simulink model "Hexalock.slx"  (R2026b)
settings: Solver=VariableStepAuto  StopTime=inf
undefined symbols (not defined in the file): gray
(part 5 of 5)

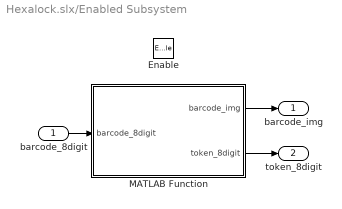
== system Hexalock.slx/Enabled Subsystem ==
  barcode_8digit : Inport
  Enable : EnablePort
  MATLAB Function : MATLAB Function  TreatAsAtomicUnit=on
  barcode_img : Outport  InitialOutput=uint8(255 * ones(80, 320))
  token_8digit : Outport  Port=2  InitialOutput=0
  wires:
  MATLAB Function/1(barcode_img) -> barcode_img/1
  MATLAB Function/2(token_8digit) -> token_8digit/1
  barcode_8digit/1 -> MATLAB Function/1(barcode_8digit)

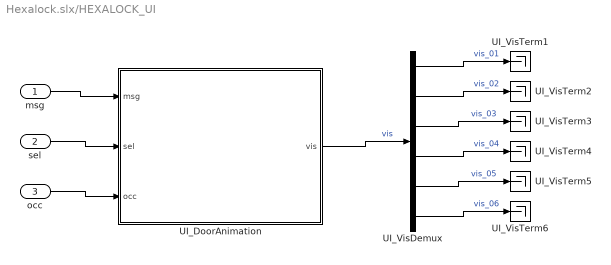
== system Hexalock.slx/HEXALOCK_UI ==
  msg : Inport
  sel : Inport  Port=2
  occ : Inport  Port=3
  UI_DoorAnimation : Stateflow chart  TreatAsAtomicUnit=on
  UI_VisDemux : Demux  Outputs=6
  UI_VisTerm{1..6} (6 alike) : Terminator
  wires:
  msg/1 -> UI_DoorAnimation/1(msg)
  sel/1 -> UI_DoorAnimation/2(sel)
  occ/1 -> UI_DoorAnimation/3(occ)
  UI_DoorAnimation/1(vis) -> UI_VisDemux/1  "vis"
  UI_VisDemux/1 -> UI_VisTerm1/1  "vis_01"
  UI_VisDemux/2 -> UI_VisTerm2/1  "vis_02"
  UI_VisDemux/3 -> UI_VisTerm3/1  "vis_03"
  UI_VisDemux/4 -> UI_VisTerm4/1  "vis_04"
  UI_VisDemux/5 -> UI_VisTerm5/1  "vis_05"
  UI_VisDemux/6 -> UI_VisTerm6/1  "vis_06"

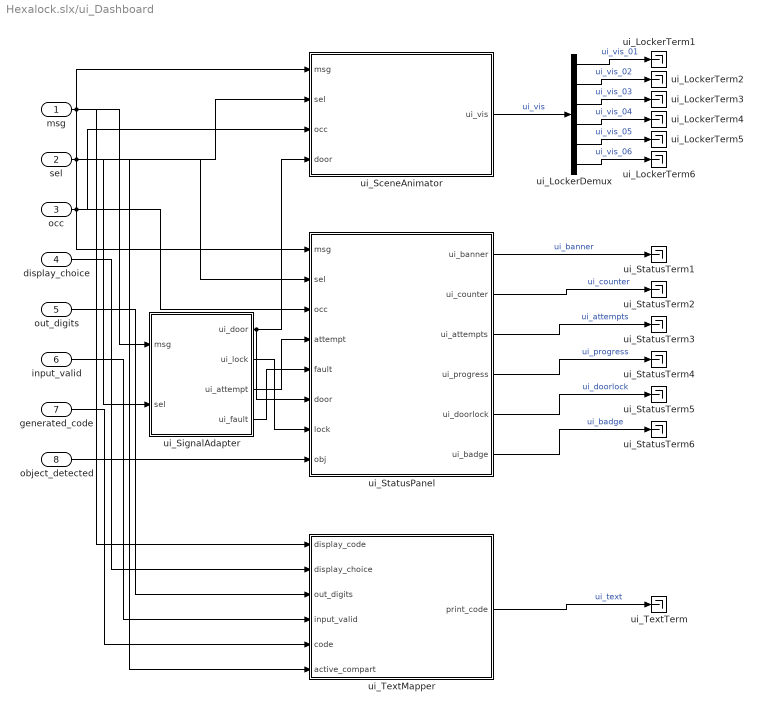
== system Hexalock.slx/ui_Dashboard ==
  msg : Inport
  sel : Inport  Port=2
  occ : Inport  Port=3
  display_choice : Inport  Port=4
  out_digits : Inport  Port=5
  input_valid : Inport  Port=6
  generated_code : Inport  Port=7
  object_detected : Inport  Port=8
  ui_LockerDemux : Demux  Outputs=6
  ui_LockerTerm{1..6} (6 alike) : Terminator
  ui_SceneAnimator : Stateflow chart  TreatAsAtomicUnit=on
  ui_SignalAdapter : Stateflow chart  TreatAsAtomicUnit=on
  ui_StatusPanel : Stateflow chart  TreatAsAtomicUnit=on
  ui_StatusTerm{1..6} (6 alike) : Terminator
  ui_TextMapper : MATLAB Function  TreatAsAtomicUnit=on
  ui_TextTerm : Terminator
  wires:
  msg/1 -> ui_SignalAdapter/1(msg), ui_SceneAnimator/1(msg), ui_StatusPanel/1(msg), ui_TextMapper/1(display_code)
  sel/1 -> ui_SignalAdapter/2(sel), ui_SceneAnimator/2(sel), ui_StatusPanel/2(sel), ui_TextMapper/6(active_compart)
  occ/1 -> ui_SceneAnimator/3(occ), ui_StatusPanel/3(occ)
  ui_SignalAdapter/1(ui_door) -> ui_SceneAnimator/4(door), ui_StatusPanel/6(door)
  ui_SceneAnimator/1(ui_vis) -> ui_LockerDemux/1  "ui_vis"
  ui_LockerDemux/1 -> ui_LockerTerm1/1  "ui_vis_01"
  ui_LockerDemux/2 -> ui_LockerTerm2/1  "ui_vis_02"
  ui_LockerDemux/3 -> ui_LockerTerm3/1  "ui_vis_03"
  ui_LockerDemux/4 -> ui_LockerTerm4/1  "ui_vis_04"
  ui_LockerDemux/5 -> ui_LockerTerm5/1  "ui_vis_05"
  ui_LockerDemux/6 -> ui_LockerTerm6/1  "ui_vis_06"
  ui_SignalAdapter/3(ui_attempt) -> ui_StatusPanel/4(attempt)
  ui_SignalAdapter/4(ui_fault) -> ui_StatusPanel/5(fault)
  ui_SignalAdapter/2(ui_lock) -> ui_StatusPanel/7(lock)
  object_detected/1 -> ui_StatusPanel/8(obj)
  ui_StatusPanel/1(ui_banner) -> ui_StatusTerm1/1  "ui_banner"
  ui_StatusPanel/2(ui_counter) -> ui_StatusTerm2/1  "ui_counter"
  ui_StatusPanel/3(ui_attempts) -> ui_StatusTerm3/1  "ui_attempts"
  ui_StatusPanel/4(ui_progress) -> ui_StatusTerm4/1  "ui_progress"
  ui_StatusPanel/5(ui_doorlock) -> ui_StatusTerm5/1  "ui_doorlock"
  ui_StatusPanel/6(ui_badge) -> ui_StatusTerm6/1  "ui_badge"
  display_choice/1 -> ui_TextMapper/2(display_choice)
  out_digits/1 -> ui_TextMapper/3(out_digits)
  input_valid/1 -> ui_TextMapper/4(input_valid)
  generated_code/1 -> ui_TextMapper/5(code)
  ui_TextMapper/1(print_code) -> ui_TextTerm/1  "ui_text"

== matlab function Hexalock.slx/Enabled Subsystem/MATLAB Function ==
  data: barcode_8digit input; barcode_img output; token_8digit output double size=1

function [barcode_img, token_8digit] = Barcode_Generator(barcode_8digit)
% Generate a Code 128C barcode for an 8-digit locker token.
% Fixed-size grayscale image: 80 rows x 320 columns.
% 0 = black, 255 = white.

barcode_img = uint8(255 * ones(80, 320));
token_8digit = barcode_8digit;
digits = zeros(1, 8);
temp = token_8digit;

for i = 8:-1:1
    digits(i) = mod(temp, 10);
    temp = floor(temp / 10);
end

% Code 128C encodes two digits per symbol.
pairs = zeros(1, 4);

for i = 1:4
    pairs(i) = digits(2*i-1)*10 + digits(2*i);
end

% Code 128 symbol patterns.
% Each row contains six alternating bar/space widths.
% Rows 1-106 correspond to symbol values 0-105.
patterns = uint8([
    2 1 2 2 2 2;
    2 2 2 1 2 2;
    2 2 2 2 2 1;
    1 2 1 2 2 3;
    1 2 1 3 2 2;
    1 3 1 2 2 2;
    1 2 2 2 1 3;
    1 2 2 3 1 2;
    1 3 2 2 1 2;
    2 2 1 2 1 3;
    2 2 1 3 1 2;
    2 3 1 2 1 2;
    1 1 2 2 3 2;
    1 2 2 1 3 2;
    1 2 2 2 3 1;
    1 1 3 2 2 2;
    1 2 3 1 2 2;
    1 2 3 2 2 1;
    2 2 3 2 1 1;
    2 2 1 1 3 2;
    2 2 1 2 3 1;
    2 1 3 2 1 2;
    2 2 3 1 1 2;
    3 1 2 1 3 1;
    3 1 1 2 2 2;
    3 2 1 1 2 2;
    3 2 1 2 2 1;
    3 1 2 2 1 2;
    3 2 2 1 1 2;
    3 2 2 2 1 1;
    2 1 2 1 2 3;
    2 1 2 3 2 1;
    2 3 2 1 2 1;
    1 1 1 3 2 3;
    1 3 1 1 2 3;
    1 3 1 3 2 1;
    1 1 2 3 1 3;
    1 3 2 1 1 3;
    1 3 2 3 1 1;
    2 1 1 3 1 3;
    2 3 1 1 1 3;
    2 3 1 3 1 1;
    1 1 2 1 3 3;
    1 1 2 3 3 1;
    1 3 2 1 3 1;
    1 1 3 1 2 3;
    1 1 3 3 2 1;
    1 3 3 1 2 1;
    3 1 3 1 2 1;
    2 1 1 3 3 1;
    2 3 1 1 3 1;
    2 1 3 1 1 3;
    2 1 3 3 1 1;
    2 1 3 1 3 1;
    3 1 1 1 2 3;
    3 1 1 3 2 1;
    3 3 1 1 2 1;
    3 1 2 1 1 3;
    3 1 2 3 1 1;
    3 3 2 1 1 1;
    3 1 4 1 1 1;
    2 2 1 4 1 1;
    4 3 1 1 1 1;
    1 1 1 2 2 4;
    1 1 1 4 2 2;
    1 2 1 1 2 4;
    1 2 1 4 2 1;
    1 4 1 1 2 2;
    1 4 1 2 2 1;
    1 1 2 2 1 4;
    1 1 2 4 1 2;
    1 2 2 1 1 4;
    1 2 2 4 1 1;
    1 4 2 1 1 2;
    1 4 2 2 1 1;
    2 4 1 2 1 1;
    2 2 1 1 1 4;
    4 1 3 1 1 1;
    2 4 1 1 1 2;
    1 3 4 1 1 1;
    1 1 1 2 4 2;
    1 2 1 1 4 2;
    1 2 1 2 4 1;
    1 1 4 2 1 2;
    1 2 4 1 1 2;
    1 2 4 2 1 1;
    4 1 1 2 1 2;
    4 2 1 1 1 2;
    4 2 1 2 1 1;
    2 1 2 1 4 1;
    2 1 4 1 2 1;
    4 1 2 1 2 1;
    1 1 1 1 4 3;
    1 1 1 3 4 1;
    1 3 1 1 4 1;
    1 1 4 1 1 3;
    1 1 4 3 1 1;
    4 1 1 1 1 3;
    4 1 1 3 1 1;
    1 1 3 1 4 1;
    1 1 4 1 3 1;
    3 1 1 1 4 1;
    4 1 1 1 3 1;
    2 1 1 4 1 2;
    2 1 1 2 1 4;
    2 1 1 2 3 2
]);

% Start Code C = 105.
% Checksum = (105 + weighted data symbols) mod 103.
checksum = 105;

for i = 1:4
    checksum = checksum + i * pairs(i);
end

checksum = mod(checksum, 103);

% Complete symbol sequence:
% Start C, 4 data pairs, checksum.
symbols = [105 pairs checksum];

% Fixed output width: 320 pixels.
% Each module is 2 pixels wide.
% Code 128C: 90 modules including stop.
% Left quiet zone begins at pixel 61.
module_width = 2;
x = 61;

% Draw six normal Code 128 symbols.
for s = 1:6
    symbol_value = symbols(s);
    widths = patterns(symbol_value + 1, :);

    for k = 1:6
        pixel_width = double(widths(k)) * module_width;

        % Odd positions represent black bars.
        if mod(k, 2) == 1
            barcode_img(9:72, x:x+pixel_width-1) = 0;
        end

        x = x + pixel_width;
    end
end

% Standard Code 128 stop pattern: 2331112.
stop_widths = [2 3 3 1 1 1 2];

for k = 1:7
    pixel_width = stop_widths(k) * module_width;

    if mod(k, 2) == 1
        barcode_img(9:72, x:x+pixel_width-1) = 0;
    end

    x = x + pixel_width;
end

end

== matlab function Hexalock.slx/MATLAB Function ==
  data: display_code input; print_code output; display_choice input; out_digits input; input_valid input; code input double size=1; active_compart input
function print_code = DisplayMapper(display_code, display_choice, out_digits, input_valid, code, active_compart)
% 1. Base prompt mapping based on system state
switch display_code
    % --- System / Idle ---
    case 0
        base_msg = "Welcome! 1#: Store | 2#: Retrieve | 333#: Maintenance";
    case 5
        base_msg = "Session timeout! Please start again";
    case 8
        base_msg = "Fault detected! Please wait for maintenance";
    case 11
        base_msg = "System locked: Attempt limit exceeded";

        % --- Store Parcel Flow ---
    case 1
        base_msg = "Select locker (1-6) + #";
    case 2
        base_msg = "Sorry, compartment unavailable";
    case 4
        base_msg = "Please place parcel";
    case 7
        base_msg = "Parcel stored! Please collect your receipt. Password:" + string(code);
    case 17
        base_msg = "Storage unavailable. All compartments are full.Please click # to return to main screen";

        % --- Retrieve Parcel Flow ---
    case 16
        base_msg = "Retrieval unavailable. All compartments are empty.Please click # to return to main screen";
    case 9
        base_msg = "Enter 6-digit PIN + #";
    case 10
        base_msg = "Error: Wrong PIN (6 digits), try again";
    case 12
        base_msg = "Please collect your parcel";
    case 13
        base_msg = "Parcel collected successfully!";
    case 26
        base_msg = "Retrieve: 11# Scan barcode | 22# Enter PIN";
    case 27
        base_msg = "Please scan your barcode";
    case 28
        base_msg = "Error: Barcode not recognised, try again";

        % --- Open & Close ---
    case 3
        base_msg = "Door " + active_compart + " opening";
    case 6
        base_msg = "Door Closing";

        % --- Maintenance Mode ---
    case 14
        base_msg = "Confirm authorisation";
    case 15
        base_msg = "To exit: confirm authorisation";
    case 18
        base_msg = "Enter Maintenance Id";
    case 19
        base_msg = "Enter Maintenance Pin";
    case 20
        base_msg = "Maintenance ID error";
    case 21
        base_msg = "Maintenance PIN error";
    case 22
        base_msg = "Maintenance Entry Successful";
    case 23
        base_msg = "MAINT ACTIVE: 1-6# Clear Box | 9# Reset All | 999# Exit";
    case 24
        base_msg = "Admin: Compartment Cleared";
    case 25
        base_msg = "Admin: All Compartments Reset!";


        % --- Default Fallback ---
    otherwise   % state 16
        base_msg = "System Ready";
end

% 2. Dynamic display rendering with input stream
if input_valid == 1
    % Instant feedback when '#' is pressed
    if out_digits > 0
        num_str = sprintf('%0*d', int64(out_digits), int64(display_choice));
        print_code = base_msg + "  [OK: " + num_str + "]";
    else
        print_code = base_msg + "  [Confirmed]";
    end

elseif out_digits > 0
    % Active typing stage: append real-time 1 to 6 digit inputs
    num_str = sprintf('%0*d', int64(out_digits), int64(display_choice));
    print_code = base_msg + "  [Input: " + num_str + "]";

else
    % Default idle or after '*' is pressed (out_digits == 0): restore clean prompt immediately
    print_code = base_msg;
end
end

== stateflow chart Hexalock.slx/Chart ==
  state Controller [parallel]
    settings: executionOrder=1
    state Main
      state StoreParcel
        state DisplayAvailable
        state OpenDoor
          en:
          lock(active_compart) = 0;
          lock_sensor(active_compart) = 0;
          motor(active_compart) = 0;
          door_sensor(active_compart) = 1;
          du:
          %Stop the motor if a fault has been detected
          if fault_detected == 1
          motor(active_compart) = 0;
          %If unlocking takes too long, stop motor and detect fault
          elseif elapsed(sec) >= 5 && ...
          lock_sensor(active_compart) ~= 0
          motor(active_compart) = 0;
          fault_detected = 1;
          %When door succesfully opens
          elseif door_sensor(active_compart) == 1
          motor(active_compart) = 0;
          %Fault detection check
          elseif door_sensor(active_compart) == 0 ||...
          lock_sensor(active_compart) == 1 ||...
          motor(active_compart) == 1;
          fault_detected = 1;
          %If it takes too long to open the door, detect fault
          elseif elapsed(sec) >= 15
          motor(active_compart) = 0;
          fault_detected = 1;
          %Turn the motor on, only after unlocking
          elseif lock_sensor(active_compart) == 0 && door_sensor(active_compart) == 0
          motor(active_compart) = 1;
          end
        state SelectCompartment
          en:
          active_compart = 0;
          du:
          if input_valid == 1 && display_choice >= 1 && display_choice <= 6
          active_compart = display_choice;
          %If locker is full, show relevant message
          if db_occupied(active_compart) == true
          outputMessage = 2;
          end
          end
        state TimeoutCloseDoor
          en:
          motor(active_compart) = -1;
          lock(active_compart) = 1;
          lock_sensor(active_compart) = 1;
          door_sensor(active_compart) = 0;
          du:
          % Stop motor if fault detected
          if fault_detected == 1
          motor(active_compart) = 0;
          %If door doesn't shut, stop motor and detect fault
          elseif elapsed(sec) >= 10 && ...
          door_sensor(active_compart) ~= 0
          motor(active_compart) = 0;
          fault_detected = 1;
          %if door is shut, stop motor and lock
          elseif door_sensor(active_compart) == 0
          motor(active_compart) = 0;
          lock(active_compart) = 1;
          %Fault detection check
          elseif door_sensor(active_compart) == 1 ||...
          lock_sensor(active_compart) == 0 ||...
          motor(active_compart) == 0;
          fault_detected = 1;
          end
          %If locking takes too long, detect fault
          if elapsed(sec) >= 5 && ...
          door_sensor(active_compart) == 0 && ...
          lock_sensor(active_compart) ~= 1
          fault_detected = 1;
          end
        state WaitForParcel
        state CloseDoor
          en:
          motor(active_compart) = -1;
          lock(active_compart) = 1;
          lock_sensor(active_compart) = 1;
          door_sensor(active_compart) = 0;
          object_sensor(active_compart) = 1;
          du:
          %Stop the motor and lock the door is closed
          if door_sensor(active_compart) == 0
          motor(active_compart) = 0;
          lock(active_compart) = 1;
          elseif door_sensor(active_compart) == 1 ||...
          lock_sensor(active_compart) == 0 ||...
          motor(active_compart) == 0;
          fault_detected = 1;
          end
          %If door doesn't shut, stop motor and detect fault
          if elapsed(sec) >= 10 && ...
          door_sensor(active_compart) ~= 0
          motor(active_compart) = 0;
          fault_detected = 1;
          outputMessage = 6;
          end
          %If locking takes too long, detect fault
          if elapsed(sec) >= 15 && ...
          door_sensor(active_compart) == 0 && ...
          lock_sensor(active_compart) ~= 1
          fault_detected = 1;
          end
          % Stop motor if fault detected
          if fault_detected == 1
          motor(active_compart) = 0;
          end
        state CheckPIN
          en:
          pin_candidate = double(random_pin);
          du:
          %Ensure the PIN isn't already used by an occupied locker in the DB
          if any((db_pins == pin_candidate) & db_occupied)
          pin_candidate = pin_candidate + 1;
          if pin_candidate > 999999
          pin_candidate = 100000;
          end
          end
        state StorageComplete
        (default) -> DisplayAvailable
        DisplayAvailable -> SelectCompartment : {outputMessage = 1;}
        SelectCompartment -> DisplayAvailable [order 1] : [after(5, sec) && active_compart >= 1 && active_compart <= 6 && ...
            |  db_occupied(active_compart) == true]
        SelectCompartment -> Controller.Main.StoreParcel.OpenDoor [order 2] : [active_compart >= 1 && active_compart <= 6 && ...
            |  db_occupied(active_compart) == false]{outputMessage = 3;}
        Controller.Main.StoreParcel.OpenDoor -> WaitForParcel : [after(2,sec) && door_sensor(active_compart) == 1 && ...
            |  lock_sensor(active_compart) == 0 && ...
            |  motor(active_compart) == 0 && ...
            |  fault_detected == 0]{outputMessage = 4;}
        WaitForParcel -> Controller.Main.StoreParcel.TimeoutCloseDoor [order 2] : [after(5,sec)]{outputMessage = 5;}
        WaitForParcel -> Controller.Main.StoreParcel.CloseDoor [order 1] : [object_detected == 1]{outputMessage = 6;}
        Controller.Main.StoreParcel.CloseDoor -> CheckPIN : [after(2,sec) && ...
            |  door_sensor(active_compart) == 0 && ...
            |  lock_sensor(active_compart) == 1 && ...
            |  motor(active_compart) == 0 && ...
            |  fault_detected == 0]
        CheckPIN -> StorageComplete : [~any((db_pins == pin_candidate) & db_occupied) && ...
            |  fault_detected == 0 && ...
            |  door_sensor(active_compart) == 0 && ...
            |  lock_sensor(active_compart) == 1 && ...
            |  motor(active_compart) == 0]
            | {generated_code = pin_candidate;
            |  store_req = true;
            |  outputMessage = 7;}
        Controller.Main.StoreParcel.TimeoutCloseDoor -> StorageComplete : [after(2, sec) && door_sensor(active_compart) == 0 && ...
            |  lock_sensor(active_compart) == 1 && ...
            |  motor(active_compart) == 0 && ...
            |  fault_detected == 0]{outputMessage = 6;}
      state Idle
        en:
        % Reset counters and selections for next user
        attempt = 0;
        active_compart = 0;
        compart_found = 0;
        fault_detected = 0;
        % Fail safe hardware enforcement
        motor = [0, 0, 0, 0, 0, 0];
        lock_sensor = [1, 1, 1, 1, 1, 1];
        door_sensor = [0, 0, 0, 0, 0, 0];
        %Display message
        outputMessage = 0;
        du:
        % Check the database: all empty = cannot retrieve, all full = cannot store
        if input_valid == 1 && display_choice == 2 && ~any(db_occupied)
        outputMessage = 16;
        elseif input_valid == 1 && display_choice == 1 && all(db_occupied)
        outputMessage = 17;
        elseif input_valid == 1
        outputMessage = 0;
        end
      state Timeout
      state RetrieveParcel
        state Enter
          outputMessage = 26;
        state CodeEntry
          en:
          compart_found = 0;
          du:
          %Pin entered
          if input_valid == 1 && out_digits == 6
          compart_found = 0;
          for i = 1:6
          if db_occupied(i) == true && display_choice == db_pins(i)
          compart_found = 1;
          active_compart = i;
          break;
          end
          end
          if compart_found == 0
          compart_found = -1;
          end
          end
        state WaitForScan
        state BarcodeEntry
          %Barcode scanned
          en:
          compart_found=0;
          du:
          if decoded_locker_id >= 1 &&...
          decoded_locker_id <= 6 && ...
          db_occupied(decoded_locker_id) == true && ...
          decoded_pin == db_pins(decoded_locker_id)
          active_compart = decoded_locker_id;
          barcode_scanned=0;
          compart_found = 1;
          end
        state InvalidCode
          en:
          attempt = attempt + 1;
          barcode_scanned = 0;
          du:
          compart_found=0;
        state Locked
        state OpenDoor
          en:
          lock(active_compart) = 0;
          lock_sensor(active_compart) = 0;
          motor(active_compart) = 0;
          door_sensor(active_compart) = 1;
          du:
          %Stop the motor if a fault has been detected
          if fault_detected == 1
          motor(active_compart) = 0;
          %If unlocking takes too long, stop motor and detect fault
          elseif elapsed(sec) >= 5 && ...
          lock_sensor(active_compart) ~= 0
          motor(active_compart) = 0;
          fault_detected = 1;
          %When door succesfully opens
          elseif door_sensor(active_compart) == 1
          motor(active_compart) = 0;
          %Fault detection check
          elseif door_sensor(active_compart) == 0 ||...
          lock_sensor(active_compart) == 1 ||...
          motor(active_compart) == 1;
          fault_detected = 1;
          %If it takes too long to open the door, detect fault
          elseif elapsed(sec) >= 15
          motor(active_compart) = 0;
          fault_detected = 1;
          %Turn the motor on, only after unlocking
          elseif lock_sensor(active_compart) == 0 && door_sensor(active_compart) == 0
          motor(active_compart) = 1;
          end
        state TimeoutCloseDoor
          en:
          motor(active_compart) = -1;
          lock(active_compart) = 1;
          lock_sensor(active_compart) = 1;
          door_sensor(active_compart) = 0;
          du:
          if fault_detected == 1
          motor(active_compart) = 0;
          elseif elapsed(sec) >= 10 && ...
          door_sensor(active_compart) ~= 0
          motor(active_compart) = 0;
          fault_detected = 1;
          elseif door_sensor(active_compart) == 0
          motor(active_compart) = 0;
          lock(active_compart) = 1;
          elseif door_sensor(active_compart) == 1 ||...
          lock_sensor(active_compart) == 0 ||...
          motor(active_compart) == 0;
          fault_detected = 1;
          end
          if elapsed(sec) >= 15 && ...
          door_sensor(active_compart) == 0 && ...
          lock_sensor(active_compart) ~= 1
          fault_detected = 1;
          end
        state WaitForRetrieval
        state CloseDoor
          en:
          motor(active_compart) = -1;
          lock(active_compart) = 1;
          lock_sensor(active_compart) = 1;
          door_sensor(active_compart) = 0;
          object_sensor(active_compart) = 0;
          du:
          %Stop the motor and lock the door is closed
          if door_sensor(active_compart) == 0
          motor(active_compart) = 0;
          lock(active_compart) = 1;
          elseif door_sensor(active_compart) == 1 ||...
          lock_sensor(active_compart) == 0 ||...
          motor(active_compart) == 0;
          fault_detected = 1;
          end
          %If door doesn't shut, stop motor and detect fault
          if elapsed(sec) >= 10 && ...
          door_sensor(active_compart) ~= 0
          motor(active_compart) = 0;
          fault_detected = 1;
          outputMessage = 6;
          end
          %If locking takes too long, detect fault
          if elapsed(sec) >= 15 && ...
          door_sensor(active_compart) == 0 && ...
          lock_sensor(active_compart) ~= 1
          fault_detected = 1;
          end
          % Stop motor if fault detected
          if fault_detected == 1
          motor(active_compart) = 0;
          end
        state RetrievalComplete
        (default) -> Enter
        Enter -> CodeEntry [order 3] : [input_valid==1&&display_choice==22]{outputMessage=9;}
        BarcodeEntry -> Enter [order 1] : [after(2,sec) && compart_found == 0]{outputMessage = 28;}
        Enter -> WaitForScan [order 1] : [input_valid==1&&display_choice==11]{outputMessage=27;}
        InvalidCode -> Enter [order 2] : [after(3,sec) && attempt<3]{outputMessage = 10;}
        WaitForScan -> BarcodeEntry [order 1] : [scanned_barcode~=0]
            | {barcode_scanned = barcode_scan(scanned_barcode);}
        CodeEntry -> InvalidCode [order 1] : [compart_found == -1||(out_digits <6 &&input_valid ==1)]
            | {outputMessage = 10;}
        CodeEntry -> Controller.Main.RetrieveParcel.OpenDoor [order 3] : [compart_found == 1]
            | {outputMessage = 3;}
        InvalidCode -> Locked [order 1] : [attempt>=3]{outputMessage = 11;}
        BarcodeEntry -> Controller.Main.RetrieveParcel.OpenDoor [order 2] : [compart_found == 1]
            | {outputMessage = 3;}
        Controller.Main.RetrieveParcel.OpenDoor -> WaitForRetrieval : [after(2,sec) && ...
            |  door_sensor(active_compart) == 1 && ...
            |  lock_sensor(active_compart) == 0 && ...
            |  motor(active_compart) == 0 && ...
            |  fault_detected == 0]{outputMessage = 12;}
        WaitForRetrieval -> Controller.Main.RetrieveParcel.TimeoutCloseDoor [order 2] : [after(5,sec)]{outputMessage = 5;}
        WaitForRetrieval -> Controller.Main.RetrieveParcel.CloseDoor [order 1] : [object_detected == 0]{outputMessage = 13;}
        Controller.Main.RetrieveParcel.TimeoutCloseDoor -> RetrievalComplete : [door_sensor(active_compart) == 0 && ...
            |  lock_sensor(active_compart) == 1 && ...
            |  motor(active_compart) == 0 && ...
            |  fault_detected == 0]{outputMessage = 6;}
        Controller.Main.RetrieveParcel.CloseDoor -> RetrievalComplete : [door_sensor(active_compart) == 0 && ...
            |  lock_sensor(active_compart) == 1 && ...
            |  motor(active_compart) == 0 && ...
            |  fault_detected == 0] ...
            | {retrieve_req = true;
            |  outputMessage = 6;}
      (default) -> Controller.Main.Idle
      SelectCompartment -> Timeout [order 3] : [after(15,sec)]{outputMessage = 5;}
      Controller.Main.Idle -> StoreParcel [order 1] : [input_valid == 1 && display_choice == 1 && ~all(db_occupied)]
      Timeout -> Controller.Main.Idle : [after(5,sec)]
      CodeEntry -> Timeout [order 2] : [after(15,sec)]{outputMessage = 5;}
      WaitForScan -> Timeout [order 2] : [after(15,sec)]{outputMessage = 5;}
      Enter -> Timeout [order 2] : [after(15,sec)]{outputMessage = 5;}
      StorageComplete -> Controller.Main.Idle : [after(2,sec) && door_sensor(active_compart) == 0 &&...
          | lock_sensor(active_compart) == 1 &&...
          | motor(active_compart) == 0]
      Locked -> Controller.Main.Idle : [after(5,sec) && ...
          |  all(door_sensor == 0) && ...
          |  all(lock_sensor == 1) && ...
          |  all(motor == 0)]
      Controller.Main.Idle -> RetrieveParcel [order 2] : [input_valid == 1 && display_choice == 2 && any(db_occupied)]
      RetrievalComplete -> Controller.Main.Idle : [after(2,sec) && all(door_sensor == 0) && ...
          |  all(lock_sensor == 1) && ...
          |  all(motor == 0)]
    state Maintanece
      state AdminActive
        en:
        maint_cmd = 0;
        maint_clear_id = 0;
        outputMessage = 23;
        confirm_active = false;
        msg_timer = 0;
        du:
        if confirm_active
        %Display confirmation message for 5 seconds
        if temporalCount(sec) - msg_timer >= 5
        outputMessage = 23;
        confirm_active = false;
        end
        elseif input_valid == 0
        maint_cmd = 0;
        maint_clear_id = 0;
        elseif input_valid == 1
        if display_choice >= 1 && display_choice <= 6
        %Target Compartment cleared
        motor(display_choice) = 0;
        lock_sensor(display_choice) = 1;
        door_sensor(display_choice) = 0;
        maint_cmd = 1;
        maint_clear_id = display_choice;
        outputMessage = 24;
        msg_timer = temporalCount(sec);
        confirm_active = true;
        elseif display_choice == 9
        %All compartment cleared
        motor = [0, 0, 0, 0, 0, 0];
        lock_sensor = [1, 1, 1, 1, 1, 1];
        door_sensor = [0, 0, 0, 0, 0, 0];
        maint_cmd = 2;
        outputMessage = 25;
        msg_timer = temporalCount(sec);
        confirm_active = true;
        elseif display_choice == 999
        %Exit Maintenance
        exit_code = true;
        end
        end
      state Idle
        du:
        is_maint = true;
        maint_cmd = 0;
        maint_clear_id = 0;
        exit_code=false;
      state VerifyAdminID
      state VerifyAdminPIN
      (default) -> Controller.Maintanece.Idle : {
          |     ADMIN_ID = 20;
          |     ADMIN_PIN = 202611;
          |     is_maint = false;
          |     maint_cmd = 0;
          |     maint_clear_id = 0;
          | }
      Controller.Maintanece.Idle -> VerifyAdminID : [input_valid == 1 &&...
          |  display_choice == 999]{outputMessage = 18}
      VerifyAdminID -> Controller.Maintanece.Idle [order 2] : [input_valid == 1 && display_choice ~= 999]
          | {outputMessage = 20;}
      VerifyAdminPIN -> AdminActive [order 1] : [input_valid == 1 &&...
          |  display_choice ==  ADMIN_PIN]{outputMessage = 22;}
      VerifyAdminID -> VerifyAdminID [order 3] : [input_valid == 1 && display_choice ~= ADMIN_ID]
          | {outputMessage = 20;}
      VerifyAdminID -> VerifyAdminPIN [order 1] : [input_valid == 1 && display_choice == ADMIN_ID]{outputMessage = 19;}
      VerifyAdminPIN -> VerifyAdminPIN [order 2] : [input_valid == 1 &&...
          |  display_choice ~=  ADMIN_PIN]{outputMessage = 21;}
    state Fault
      en:
      motor(:) = 0;
      outputMessage = 8;
    (default) -> Main
    Maintanece -> Main : [exit_code == true && all(door_sensor == 0) && all(lock_sensor == 1) && all(motor == 0)]
        | {fault_detected = 0; exit_code = false; is_maint = false;}
    Main -> Maintanece [order 1] : [input_valid == 1 && display_choice == 333 && all(door_sensor == 0) && all(lock_sensor == 1) && all(motor == 0)]{outputMessage = 14;}
    Fault -> Maintanece : [display_choice == 333 ]{outputMessage = 14;}
    Main -> Fault [order 2] : [fault_detected==1]{outputMessage = 8;}
  state DB [parallel]
    settings: executionOrder=3
    state Barcode_Decoder [parallel]
      entry:
      decoded_locker_id = 0;
      decoded_pin = 0;
      during:
      %Decode when the database middleware confirms the scanned barcode exists
      if decode_en == 1 && barcode_scanned >= 30000000 && barcode_scanned <= 39999999
      M = 10000000;
      B = 7391258;
      cipher_val = double(barcode_scanned) - 30000000;
      %Inverse of hash
      raw_combined = mod(B - cipher_val, M);
      decoded_locker_id = floor(raw_combined / 1000000);
      decoded_pin = mod(raw_combined, 1000000);
      else
      decoded_locker_id = 0;
      decoded_pin = 0;
      end
      settings: executionOrder=1
    state Barcode_Encoder [parallel]
      en:
      barcode_8digit = 0;
      du:
      if outputMessage == 7 && (active_compart >= 1 && active_compart <= 6) && (generated_code >= 100000 && generated_code <= 999999)
      M = 10000000;
      B = 7391258;
      raw_combined = double(active_compart) * 1000000 + double(generated_code);
      cipher_val = mod(B - raw_combined, M);
      barcode_8digit = 30000000 + cipher_val;
      barcode_scan(active_compart) = barcode_8digit;
      else
      barcode_8digit = 0;
      end
      settings: executionOrder=2
    state DB_Middleware [parallel]
      en:
      %0: Idle, 1: Store Write, 2: Retrieve Clear, 3: Admin Single Clear, 4: Admin All Reset
      db_cmd = 0;
      db_target_id = 0;
      db_new_barcode = 0;
      db_new_pin = 0;
      decode_en = 0;
      lost_verify_ok = 0;
      lost_check_req = false;
      req_locker_id = 0;
      req_pin = 0;
      du:
      %Reset database values after each step
      db_cmd = 0;
      db_target_id = 0;
      db_new_barcode = 0;
      db_new_pin = 0;
      decode_en = 0;
      lost_verify_ok = 0;
      %Maintenance logic
      if is_maint == true || fault_detected == 1
      if maint_cmd == 1 && (maint_clear_id >= 1 && maint_clear_id <= 6)
      db_cmd = 3;
      db_target_id = maint_clear_id;
      elseif maint_cmd == 2
      db_cmd = 4;
      end
      else
      %Stores request from main
      if store_req == true && (active_compart >= 1 && active_compart <= 6) && barcode_8digit >= 30000000
      db_cmd = 1;
      db_target_id = active_compart;
      db_new_pin = generated_code;
      db_new_barcode = barcode_8digit;
      store_req = false;
      %Retrieves request from main
      elseif retrieve_req == true && (active_compart >= 1 && active_compart <= 6)
      db_cmd = 2;
      db_target_id = active_compart;
      retrieve_req = false;
      %Check the scanned barcode exists
      elseif barcode_scanned >= 30000000 && barcode_scanned <= 39999999
      for i = 1:6
      if db_occupied(i) == true && db_barcode(i) == barcode_scanned
      decode_en = 1;
      break;
      end
      end
      %Match the barcode if user lost recipt
      elseif lost_check_req == true && (req_locker_id >= 1 && req_locker_id <= 6) && (req_pin >= 100000 && req_pin <= 999999)
      re_raw = double(req_locker_id) * 1000000 + double(req_pin);
      re_barcode = 30000000 + mod(7391258 - re_raw, 10000000);
      if db_occupied(req_locker_id) == true && db_barcode(req_locker_id) == re_barcode
      lost_verify_ok = 1;
      end
      end
      end
      settings: executionOrder=3
    state DataBase_Core [parallel]
      entry:
      db_occupied = [false false false false false false];
      db_locked   = [true true true true true true];
      db_barcode  = [0 0 0 0 0 0];
      db_pins     = [0 0 0 0 0 0];
      during:
      %Compartment doors remain locked
      if is_maint == true || fault_detected == 1
      db_locked   = [true true true true true true];
      door_sensor = [0 0 0 0 0 0];
      motor       = [0 0 0 0 0 0];
      end
      switch db_cmd
      case 1 %Store
      db_occupied(db_target_id) = true;
      db_barcode(db_target_id)  = db_new_barcode;
      db_pins(db_target_id)     = db_new_pin;
      case 2 %Retrieve
      db_occupied(db_target_id) = false;
      db_barcode(db_target_id)  = 0;
      db_pins(db_target_id)     = 0;
      case 3 %Clear one compartment
      db_occupied(db_target_id) = false;
      db_barcode(db_target_id)  = 0;
      db_pins(db_target_id)     = 0;
      case 4 %Reset all compartments
      db_occupied = [false false false false false false];
      db_barcode  = [0 0 0 0 0 0];
      db_pins     = [0 0 0 0 0 0];
      end
      compart_availability = double(db_occupied);
      code = db_pins;
      settings: executionOrder=4
    (default) -> DB_Middleware [order 1]
    (default) -> DataBase_Core [order 2]
  state Buffer [parallel]
    en:
    buffer = 0;
    digit_count = 0;
    input_valid = 0;
    last_key = -1;
    du:
    if input_valid == 1
    input_valid = 0;
    buffer = 0;
    digit_count = 0;
    end
    %Checking for keypad spammed entry
    if keypad_input ~= last_key && keypad_input ~= -1
    %Checking if keypad entry is from 0 to 9
    if keypad_input >= 0 && keypad_input <= 9
    % Limits input to 6 digits
    if digit_count < 6
    buffer = buffer * 10 + keypad_input;
    digit_count = digit_count + 1;
    end
    input_valid = 0;
    %Clear input upon pressing *
    elseif keypad_input == 11
    buffer = 0;
    digit_count = 0;
    input_valid = 0;
    %Confirm input upon pressing #
    elseif keypad_input == 12
    input_valid = 1;
    end
    end
    %Output sent to a main controller and display mapper
    display_choice = buffer;
    out_digits = digit_count;
    last_key = keypad_input;
    settings: executionOrder=2
  (default) -> DB
  data: attempt local double size=1 =0; motor local double size=[1 6] =zeros(1, 6); lock local double size=[1 6] =ones(1, 6); compart_found local double size=1 =0; door_sensor local double size=[1 6] =zeros(1, 6); lock_sensor local double size=[1 6] =ones(1, 6); outputMessage output size=1; fault_detected local double size=1 =0; keypad_input input; input_valid output =0; out_digits output =0; display_choice output =0; digit_count local; buffer local; last_key local; object_sensor local double size=[1 6] =zeros(1, 6); object_detected input; code local double size=[1 6] =zeros(1, 6); i local; active_compart output double size=1 =0; generated_code output double =0; random_pin input uint32 size=1; pin_candidate local double size=1 =0; ADMIN_ID local; ADMIN_PIN local; exit_code local boolean size=1 =false; B local double size=1 =7391258; M local double size=1 =10000000; cipher_val local double size=1 =0; db_barcode local double size=[1 6] =zeros(1,6); db_cmd local double size=1 =0; db_new_barcode local double size=1 =0; db_new_pin local double =0; db_occupied local boolean size=[1 6] =false(1,6); db_target_id local double size=1 =0; decode_en local double size=1 =0; lost_check_req local boolean size=1 =false; raw_combined local double size=1 =0; re_barcode local double size=1 =0; re_raw local double size=1 =0; req_locker_id local double size=1 =0; req_pin local double size=1 =0; decoded_locker_id local double size=1 =0; decoded_pin local double size=1 =0; lost_verify_ok local double size=1 =0; maint_cmd local; maint_clear_id local; is_maint local boolean size=1 =false; db_locked local boolean size=[1 6] =true(1,6); db_pins local double size=[1 6] =zeros(1,6); retrieve_req local boolean size=1 =false; store_req local boolean size=1 =false; compart_availability output double size=[1 6] =zeros(1, 6); confirm_active local boolean size=1 =false; msg_timer local double size=1 =0; barcode_8digit output double size=1 =0; barcode_scan data_store_memory size=1 =0; scanned_barcode input double size=1; barcode_scanned data_store_memory size=1

== stateflow chart Hexalock.slx/HEXALOCK_UI/UI_DoorAnimation ==
  settings: description=Display-only door animation and visual-code renderer. Not part of the access-control logic.
  state UI_Door [parallel]
    settings: executionOrder=1
    state UI_Opening1
      en: frame = 4;
    state UI_Opening2
      en: frame = 5;
    state UI_Opening3
      en: frame = 6;
    state UI_Open
      en: frame = 7;
    state UI_Closed
      en:
      frame = 0;
      door_idx = 0;
    state UI_Closing3
      en: frame = 10;
    state UI_Closing2
      en: frame = 9;
    state UI_Closing1
      en: frame = 8;
    (default) -> UI_Closed
    UI_Closed -> UI_Opening1 : [msg == 3 && prev_msg ~= 3 && ...
        |  sel >= 1 && sel <= 6]
        | {door_idx = sel;}
    UI_Opening1 -> UI_Opening2 : [after(0.2,sec)]
    UI_Opening2 -> UI_Opening3 : [after(0.2,sec)]
    UI_Opening3 -> UI_Open : [after(0.2,sec)]
    UI_Open -> UI_Closing1 : [msg == 5 || msg == 6 || ...
        |  msg == 13 || sel == 0]
    UI_Closing3 -> UI_Closed : [after(0.2,sec)]
    UI_Closing2 -> UI_Closing3 : [after(0.2,sec)]
    UI_Closing1 -> UI_Closing2 : [after(0.2,sec)]
  state UI_Render [parallel]
    en, du:
    for k = 1:6
    if frame > 0 && k == door_idx
    vis(k) = frame;
    elseif msg == 23 || msg == 24 || msg == 25
    vis(k) = 11;
    else
    vis(k) = double(occ(k) ~= 0) + 2 * double(sel == k);
    end
    end
    prev_msg = msg;
    settings: executionOrder=2
  data: msg input; sel input; occ input size=[1 6]; vis output double size=[1 6] =zeros(1, 6); door_idx local double =0; frame local double =0; prev_msg local double =-1; k local double =0

== stateflow chart Hexalock.slx/ui_Dashboard/ui_SceneAnimator ==
  settings: description=Display-only parcel/door animation. Inputs are read-only copies of controller outputs.
  state ui_Events [parallel]
    en, du:
    % one-step event flags from controller outputs
    ui_rise = 0;
    ui_fall = 0;
    for ui_i = 1:6
    if door(ui_i) ~= 0 && ui_prev_door(ui_i) == 0
    ui_rise = ui_i;
    end
    if door(ui_i) == 0 && ui_prev_door(ui_i) ~= 0
    ui_fall = ui_i;
    end
    end
    % placement accepted: msg 4 -> 6, removal accepted: msg 12 -> 13
    ui_place = double(ui_prev_msg == 4 && msg == 6);
    ui_remove = double(ui_prev_msg == 12 && msg == 13);
    ui_prev_door = door;
    ui_prev_msg = msg;
    settings: executionOrder=1
  state ui_Sequencer [parallel]
    settings: executionOrder=2
    state ui_Idle
      en:
      ui_frame = 0;
      ui_k = 0;
    state ui_Active
      state ui_DoorOpen
        en:
        if ui_obase == 36
        ui_frame = 26;
        else
        ui_frame = 20;
        end
      state ui_Opening
        en, du:
        ui_frame = ui_obase + ...
        min(floor(temporalCount(sec) / 0.2), 2);
      state ui_Collecting
        en, du:
        ui_n = floor(temporalCount(sec) / 0.15);
        if ui_n <= 4
        ui_frame = 27 + ui_n;
        else
        ui_frame = 32;
        end
      state ui_Placing
        en, du:
        ui_n = floor(temporalCount(sec) / 0.15);
        if ui_n <= 4
        ui_frame = 21 + ui_n;
        else
        ui_frame = 26;
        end
      state ui_Closing
        en, du:
        ui_frame = ui_cbase + ...
        min(floor(temporalCount(sec) / 0.2), 2);
      (default) -> ui_Opening
      ui_Active -> ui_Active : [ui_rise > 0]
          | {ui_k = ui_rise;
          |  ui_obase = 4 + 32 * double(occ(ui_rise) ~= 0);}
      ui_Opening -> ui_DoorOpen [order 4] : [after(0.6, sec)]
      ui_DoorOpen -> ui_Placing [order 1] : [ui_place > 0]
      ui_DoorOpen -> ui_Closing [order 3] : [ui_fall == ui_k]
          | {ui_cbase = 8 + 25 * double(occ(ui_k) ~= 0);}
      ui_DoorOpen -> ui_Collecting [order 2] : [ui_remove > 0]
      ui_Opening -> ui_Collecting [order 2] : [ui_remove > 0]
      ui_Opening -> ui_Closing [order 3] : [ui_fall == ui_k]
          | {ui_cbase = 8 + 25 * double(occ(ui_k) ~= 0);}
      ui_Opening -> ui_Placing [order 1] : [ui_place > 0]
      ui_Collecting -> ui_Closing : [after(1.05, sec)]
          | {ui_cbase = 8;}
      ui_Placing -> ui_Closing : [after(1.05, sec)]
          | {ui_cbase = 33;}
    (default) -> ui_Idle
    ui_Idle -> ui_Active : [ui_rise > 0]
        | {ui_k = ui_rise;
        |  ui_obase = 4 + 32 * double(occ(ui_rise) ~= 0);}
    ui_Closing -> ui_Idle : [after(0.6, sec)]
  state ui_Render [parallel]
    en, du:
    for ui_i = 1:6
    if ui_frame > 0 && ui_i == ui_k
    ui_vis(ui_i) = ui_frame;
    elseif msg == 23 || msg == 24 || msg == 25
    ui_vis(ui_i) = 11;
    else
    ui_vis(ui_i) = double(occ(ui_i) ~= 0) + 2 * double(sel == ui_i);
    end
    end
    settings: executionOrder=3
  data: msg input; sel input; occ input size=[1 6]; door input size=[1 6]; ui_vis output double size=[1 6] =zeros(1, 6); ui_k local double =0; ui_frame local double =0; ui_rise local double =0; ui_fall local double =0; ui_place local double =0; ui_remove local double =0; ui_i local double =0; ui_n local double =0; ui_prev_msg local double =-1; ui_prev_door local double size=[1 6] =zeros(1, 6); ui_obase local double =4; ui_cbase local double =8

== stateflow chart Hexalock.slx/ui_Dashboard/ui_StatusPanel ==
  settings: description=Display-only status derivation (banner, counter, attempts, progress, door/lock, parcel sensor).
  state ui_Mode [parallel]
    en, du:
    % maintenance messages are only issued by Maintanece
    ui_maint = double(msg == 14 || (msg >= 18 && msg <= 25));
    settings: executionOrder=1
  state ui_Sensors [parallel]
    en, du:
    ui_doorlock = 0;
    if sel >= 1 && sel <= 6
    if door(sel) == 0 && lock(sel) ~= 0
    ui_doorlock = 1;
    elseif door(sel) == 0
    ui_doorlock = 2;
    elseif lock(sel) == 0
    ui_doorlock = 3;
    else
    ui_doorlock = 4;
    end
    end
    if obj == 1
    ui_badge = 1;
    elseif obj == 0
    ui_badge = 2;
    else
    ui_badge = 0;
    end
    settings: executionOrder=5
  state ui_Progress [parallel]
    settings: executionOrder=6
    state ui_PIdle
      en, du:
      ui_kind = 0;
      ui_stage = 0;
      if ui_maint == 1
      ui_progress = 50;
      else
      ui_progress = 0;
      end
    state ui_PHold
      % keep the one-step retrieval result visible
    state ui_PTrack
      en, du:
      switch msg
      case {1, 2}
      ui_kind = 1;
      ui_progress = 11;
      case {9, 10, 26, 27, 28}
      ui_kind = 2;
      ui_progress = 21;
      case 11
      ui_progress = 27;
      case {3, 4}
      if ui_kind == 2
      ui_progress = 22;
      else
      ui_progress = 12;
      end
      case 12
      ui_progress = 22;
      case 13
      ui_progress = 23;
      case 5
      if ui_kind == 2
      ui_progress = 25;
      else
      ui_progress = 15;
      end
      case 6
      if ui_kind == 2
      if ui_progress == 25 || ui_progress == 26
      ui_progress = 26;
      else
      ui_progress = 24;
      end
      elseif ui_progress == 15 || ui_progress == 16
      ui_progress = 16;
      else
      ui_progress = 13;
      end
      case 7
      ui_progress = 14;
      case 8
      if ui_progress < 30
      if ui_kind == 1
      if ui_progress >= 15
      ui_stage = 3;
      else
      ui_stage = ui_progress - 10;
      end
      ui_progress = 30 + ui_stage;
      elseif ui_kind == 2
      if ui_progress == 27
      ui_stage = 1;
      elseif ui_progress >= 25
      ui_stage = 3;
      else
      ui_stage = ui_progress - 20;
      end
      ui_progress = 40 + ui_stage;
      else
      ui_progress = 30;
      end
      end
      end
    (default) -> ui_PIdle
    ui_PHold -> ui_PIdle : [after(2, sec) || msg ~= 0]
    ui_PTrack -> ui_PHold [order 1] : [msg == 0 && (ui_progress == 24 || ui_progress == 26)]
    ui_PIdle -> ui_PTrack : [msg == 1 || msg == 26 || msg == 9 || msg == 8]
    ui_PTrack -> ui_PIdle [order 2] : [msg == 0 || msg == 16 || msg == 17 || ui_maint == 1]
  state ui_Banner [parallel]
    en, du:
    if msg == 8
    ui_banner = 3;
    elseif ui_maint == 1
    if fault == 1
    ui_banner = 5;
    elseif msg >= 22
    ui_banner = 2;
    else
    ui_banner = 1;
    end
    elseif fault == 1
    ui_banner = 3;
    elseif msg == 11
    ui_banner = 4;
    else
    ui_banner = 0;
    end
    settings: executionOrder=2
  state ui_Counter [parallel]
    en, du:
    ui_counter = sum(double(occ ~= 0));
    settings: executionOrder=3
  state ui_Attempts [parallel]
    en, du:
    % limit 3 = controller guard [attempt >= 3]
    if msg == 9 || msg == 10 || msg == 26 || msg == 27 || msg == 28
    if attempt >= 3
    ui_attempts = 4;
    else
    ui_attempts = 3 - attempt;
    end
    elseif msg == 11
    ui_attempts = 4;
    else
    ui_attempts = 0;
    end
    settings: executionOrder=4
  data: msg input; sel input; occ input size=[1 6]; attempt input; fault input; door input size=[1 6]; lock input size=[1 6]; obj input; ui_banner output double =0; ui_counter output double =0; ui_attempts output double =0; ui_progress output double =0; ui_doorlock output double =0; ui_badge output double =0; ui_maint local double =0; ui_kind local double =0; ui_stage local double =0

== matlab function Hexalock.slx/ui_Dashboard/ui_TextMapper ==
  data: display_code input; print_code output; display_choice input; out_digits input; input_valid input; code input; active_compart input
function print_code = ui_TextMapper(display_code, display_choice, out_digits, input_valid, code, active_compart)
% UI-only: digits typed at a PIN prompt (msg 9 = customer PIN, 19/21 = admin PIN)
% are echoed as '*'. Menu choices, locker numbers and the admin ID stay readable.
% The prompt showing when typing began is latched, so the mask cannot drop mid-entry.
persistent ui_ctx
if isempty(ui_ctx)
    ui_ctx = -1;
end
if out_digits == 0 && input_valid == 0
    ui_ctx = display_code;
end
ui_mask = ui_is_pin_prompt(display_code) || ui_is_pin_prompt(ui_ctx);

% 1. Base prompt mapping based on system state
switch display_code
    % --- System / Idle ---
    case 0
        base_msg = "Welcome! 1#: Store | 2#: Retrieve | 333#: Maintenance";
    case 5
        base_msg = "Session timeout! Please start again";
    case 8
        base_msg = "Fault detected! Please wait for maintenance";
    case 11
        base_msg = "System locked: Attempt limit exceeded";

        % --- Store Parcel Flow ---
    case 1
        base_msg = "Select locker (1-6) + #";
    case 2
        base_msg = "Sorry, compartment unavailable";
    case 4
        base_msg = "Please place parcel";
    case 7
        base_msg = "Parcel stored! Please collect your receipt. Password:" + string(code);
    case 17
        base_msg = "Storage unavailable. All compartments are full.Please click # to return to main screen";

        % --- Retrieve Parcel Flow ---
    case 16
        base_msg = "Retrieval unavailable. All compartments are empty.Please click # to return to main screen";
    case 9
        base_msg = "Enter 6-digit PIN + #";
    case 10
        base_msg = "Error: Wrong PIN (6 digits), try again";
    case 12
        base_msg = "Please collect your parcel";
    case 13
        base_msg = "Parcel collected successfully!";
    case 26
        base_msg = "Retrieve: 11# Scan barcode | 22# Enter PIN";
    case 27
        base_msg = "Please scan your barcode";
    case 28
        base_msg = "Error: Barcode not recognised, try again";

        % --- Open & Close ---
    case 3
        base_msg = "Door " + active_compart + " opening";
    case 6
        base_msg = "Door Closing";

        % --- Maintenance Mode ---
    case 14
        base_msg = "Confirm authorisation";
    case 15
        base_msg = "To exit: confirm authorisation";
    case 18
        base_msg = "Enter Maintenance Id";
    case 19
        base_msg = "Enter Maintenance Pin";
    case 20
        base_msg = "Maintenance ID error";
    case 21
        base_msg = "Maintenance PIN error";
    case 22
        base_msg = "Maintenance Entry Successful";
    case 23
        base_msg = "MAINT ACTIVE: 1-6# Clear Box | 9# Reset All | 999# Exit";
    case 24
        base_msg = "Admin: Compartment Cleared";
    case 25
        base_msg = "Admin: All Compartments Reset!";


        % --- Default Fallback ---
    otherwise   % state 16
        base_msg = "System Ready";
end

% 2. Dynamic display rendering with input stream
if input_valid == 1
    % Instant feedback when '#' is pressed
    if out_digits > 0
        num_str = ui_echo(display_choice, out_digits, ui_mask);
        print_code = base_msg + "  [OK: " + num_str + "]";
    else
        print_code = base_msg + "  [Confirmed]";
    end

elseif out_digits > 0
    % Active typing stage: append real-time 1 to 6 digit inputs
    num_str = ui_echo(display_choice, out_digits, ui_mask);
    print_code = base_msg + "  [Input: " + num_str + "]";

else
    % Default idle or after '*' is pressed (out_digits == 0): restore clean prompt immediately
    print_code = base_msg;
end
end

function tf = ui_is_pin_prompt(c)
tf = (c == 9 || c == 19 || c == 21);
end

function s = ui_echo(v, n, masked)
if masked
    s = repmat('*', 1, max(0, round(double(n))));
else
    s = sprintf('%0*d', int64(n), int64(v));
end
end

== stateflow chart Hexalock.slx/ui_Dashboard/ui_SignalAdapter ==
  settings: description=Display-only. Reconstructs the door/lock state, attempt count and fault flag that the controller sets alongside each outputMessage, using outputMessage and active_compart only.
  state ui_Derive
    en, du:
    if msg ~= ui_prev_msg
    % door opening (msg 3) / door closing (msg 5, 6, 13) on the active compartment
    if msg == 3 && sel >= 1 && sel <= 6
    ui_door(sel) = 1;
    ui_lock(sel) = 0;
    elseif (msg == 5 || msg == 6 || msg == 13) && sel >= 1 && sel <= 6
    ui_door(sel) = 0;
    ui_lock(sel) = 1;
    elseif msg == 8
    % fault: DB_Core forces every door closed
    ui_door = zeros(1, 6);
    ui_fault = 1;
    elseif msg == 25
    ui_lock = ones(1, 6);
    end
    % InvalidCode is entered with msg 10 from CodeEntry (msg 9) or msg 28 from BarcodeEntry
    if (ui_prev_msg == 9 && msg == 10) || msg == 28
    ui_attempt = ui_attempt + 1;
    end
    end
    % Main/Idle entry (msg 0) resets doors, locks, attempt and fault
    if msg == 0
    ui_door = zeros(1, 6);
    ui_lock = ones(1, 6);
    ui_attempt = 0;
    ui_fault = 0;
    end
    ui_prev_msg = msg;
  (default) -> ui_Derive
  data: msg input; sel input; ui_door output double size=[1 6] =zeros(1, 6); ui_lock output double size=[1 6] =ones(1, 6); ui_attempt output double =0; ui_fault output double =0; ui_prev_msg local double =-1
